simulink model "gnc_SpeedGovernor"  (R2026b)
settings: Solver=VariableStepAuto
values from neighbouring files (symbols this model uses):
  Ts = prm.Ts    [gnc_missionFSM.m]    (also in gnc_mpcPlantUpdate.m)
undefined symbols (not defined in the file or in its folder): P
libraries: sl_discontinuities x1, simulink x1
settings Model: Creator=aomar  LastModifiedBy=aomar

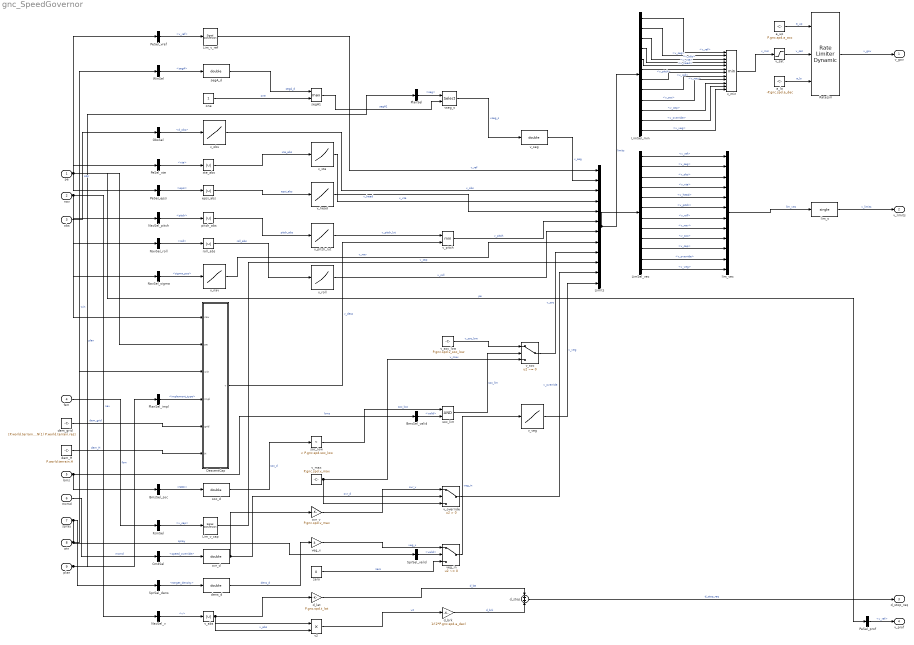
== system gnc_SpeedGovernor ==
  pe : Inport  OutDataTypeStr=Bus: Bus_PathError  SampleTime=Ts.gnc
  nav : Inport  Port=2  OutDataTypeStr=Bus: Bus_NavCond  SampleTime=Ts.gnc
  obs : Inport  Port=3  OutDataTypeStr=Bus: Bus_ObsFlags  SampleTime=Ts.gnc
  fsm : Inport  Port=4  OutDataTypeStr=Bus: Bus_FsmOut  SampleTime=Ts.gnc
  bms : Inport  Port=5  OutDataTypeStr=Bus: Bus_BmsStatus  SampleTime=Ts.gnc
  mcmd : Inport  Port=6  OutDataTypeStr=Bus: Bus_MissionCmd  SampleTime=Ts.gnc
  spray : Inport  Port=7  OutDataTypeStr=Bus: Bus_SprayDemand  SampleTime=Ts.gnc
  win : Inport  Port=8  OutDataTypeStr=Bus: Bus_PathWindow  SampleTime=Ts.gnc
  plan : Inport  Port=9  OutDataTypeStr=Bus: Bus_MissionPlan
  BmsSel_soc : BusSelector  OutputSignals=SOC
  BmsSel_valid : BusSelector  OutputSignals=valid
  CmdSel : BusSelector  OutputSignals=speed_override
  DescentCap : MATLAB Function  TreatAsAtomicUnit=on  mask{desc=P.gnc.desc}
  FsmSel : BusSelector  OutputSignals=v_cap
  LimSel_min : BusSelector  OutputSignals=v_ref,v_seg,v_obs,v_xte,v_head,v_pitch,v_roll,v_nav,v_soc,v_cap,v_override,v_veg
  LimSel_vec : BusSelector  OutputSignals=v_ref,v_seg,v_obs,v_xte,v_head,v_pitch,v_roll,v_nav,v_soc,v_cap,v_override,v_veg
  Lim_v_cap : SignalConversion  OverrideOpt=off
  Lim_v_ref : SignalConversion  OverrideOpt=off
  Limits : BusCreator  Inputs=12
  NavSel_pitch : BusSelector  OutputSignals=pitch
  NavSel_roll : BusSelector  OutputSignals=roll
  NavSel_sigma : BusSelector  OutputSignals=sigma_pos
  NavSel_v : BusSelector  OutputSignals=v
  ObsSel : BusSelector  OutputSignals=d_obs
  PeSel_epsi : BusSelector  OutputSignals=epsi
  PeSel_prof : BusSelector  OutputSignals=v_ref
  PeSel_vref : BusSelector  OutputSignals=v_ref
  PeSel_xte : BusSelector  OutputSignals=xte
  PlanSel : BusSelector  OutputSignals=seg
  PlanSel_impl : BusSelector  OutputSignals=implement_type
  RateLim : sl_discontinuities/Rate Limiter Dynamic
      settings: LibrarySourceBlock=|
      | simulink/Discontinuities/Rate Limiter
      | Dynamic
  SprSel_dens : BusSelector  OutputSignals=target_density
  SprSel_valid : BusSelector  OutputSignals=valid
  WinSel : BusSelector  OutputSignals=segA
  a_lo : Constant  Value=-P.gnc.spd.a_dec  OutDataTypeStr=double  SampleTime=Ts.gnc
  a_up : Constant  Value=P.gnc.spd.a_acc  OutDataTypeStr=double  SampleTime=Ts.gnc
  d_brk : Gain  Gain=1/(2*P.gnc.spd.a_dec)
  d_lat : Gain  Gain=P.gnc.spd.t_lat
  d_stop : Sum
  dem_H : Constant  Value=P.world.terrain.H  OutDataTypeStr=double
  dem_grid : Constant  Value=[P.world.terrain.xE(1) P.world.terrain.yN(1) P.world.terrain.res]  OutDataTypeStr=double
  dens_d : DataTypeConversion  OutDataTypeStr=double  RndMeth=Nearest
  epsi_abs : Abs  SaturateOnIntegerOverflow=off
  lim_s : DataTypeConversion  OutDataTypeStr=single  RndMeth=Nearest
  lim_vec : Mux  Inputs=12
  one : Constant  OutDataTypeStr=double  SampleTime=Ts.gnc
  ovr_d : DataTypeConversion  OutDataTypeStr=double  RndMeth=Nearest
  ovr_v : Gain  Gain=P.gnc.spd.v_max
  pitch_abs : Abs  SaturateOnIntegerOverflow=off
  roll_abs : Abs  SaturateOnIntegerOverflow=off
  segA1 : MinMax  Function=max  Inputs=2
  segA_d : DataTypeConversion  OutDataTypeStr=double  RndMeth=Nearest
  soc_d : DataTypeConversion  OutDataTypeStr=double  RndMeth=Nearest
  soc_lim : Logic  AllPortsSameDT=off  OutDataTypeStr=boolean
  soc_low : simulink/Logic and Bit Operations/Compare To Constant  relop=<  const=P.gnc.spd.soc_low  OutDataTypeStr=boolean
  v2 : Product  Inputs=**
  v_abs : Abs  SaturateOnIntegerOverflow=off
  v_head : Lookup_n-D  NumberOfTableDimensions=1  BreakpointsForDimension1=P.gnc.spd.head_x  Table=P.gnc.spd.head_v  ExtrapMethod=Clip  UseLastTableValue=on  InternalRulePriority=Speed  RndMeth=Simplest
  v_max : Constant  Value=P.gnc.spd.v_max  OutDataTypeStr=double  SampleTime=Ts.gnc
  v_min : MinMax  Inputs=12
  v_nav : Lookup_n-D  NumberOfTableDimensions=1  BreakpointsForDimension1=P.gnc.spd.nav_x  Table=P.gnc.spd.nav_v  ExtrapMethod=Clip  UseLastTableValue=on  InternalRulePriority=Speed  RndMeth=Simplest
  v_obs : Lookup_n-D  NumberOfTableDimensions=1  BreakpointsForDimension1=P.gnc.spd.obs_d  Table=P.gnc.spd.obs_v  ExtrapMethod=Clip  UseLastTableValue=on  InternalRulePriority=Speed  RndMeth=Simplest
  v_override : Switch  Criteria=u2 > Threshold  SaturateOnIntegerOverflow=off  InputSameDT=off
  v_pitch : MinMax  Inputs=2
  v_pitch_lut : Lookup_n-D  NumberOfTableDimensions=1  BreakpointsForDimension1=P.gnc.spd.pitch_x  Table=P.gnc.spd.pitch_v  ExtrapMethod=Clip  UseLastTableValue=on  InternalRulePriority=Speed  RndMeth=Simplest
  v_roll : Lookup_n-D  NumberOfTableDimensions=1  BreakpointsForDimension1=P.gnc.spd.roll_x  Table=P.gnc.spd.roll_v  ExtrapMethod=Clip  UseLastTableValue=on  InternalRulePriority=Speed  RndMeth=Simplest
  v_sat : Saturate  UpperLimit=P.gnc.spd.v_max  LowerLimit=0
  v_seg : DataTypeConversion  OutDataTypeStr=double  RndMeth=Nearest
  v_soc : Switch  Criteria=u2 ~= 0  SaturateOnIntegerOverflow=off  InputSameDT=off
  v_soc_low : Constant  Value=P.gnc.spd.v_soc_low  OutDataTypeStr=double  SampleTime=Ts.gnc
  v_veg : Lookup_n-D  NumberOfTableDimensions=1  BreakpointsForDimension1=P.gnc.spd.veg_x  Table=P.gnc.spd.veg_v  ExtrapMethod=Clip  UseLastTableValue=on  InternalRulePriority=Speed  RndMeth=Simplest
  v_xte : Lookup_n-D  NumberOfTableDimensions=1  BreakpointsForDimension1=P.gnc.spd.xte_x  Table=P.gnc.spd.xte_v  ExtrapMethod=Clip  UseLastTableValue=on  InternalRulePriority=Speed  RndMeth=Simplest
  veg_in : Switch  Criteria=u2 ~= 0  SaturateOnIntegerOverflow=off  InputSameDT=off
  veg_x : Gain  Gain=3
  vseg_s : Selector  NumberOfDimensions=2  InputPortWidth=3  IndexOptions=Index vector (port),Index vector (dialog)  Indices=1,4  OutputSizes=1
  xte_abs : Abs  SaturateOnIntegerOverflow=off
  zero : Constant  Value=0  OutDataTypeStr=double  SampleTime=Ts.gnc
  v_gov : Outport  OutDataTypeStr=double
  v_limits : Outport  Port=2  OutDataTypeStr=single
  d_stop_req : Outport  Port=3  OutDataTypeStr=double
  v_prof : Outport  Port=4  OutDataTypeStr=double
  wires:
  obs/1 -> ObsSel/1  "obs"
  fsm/1 -> FsmSel/1  "fsm"
  dem_grid/1 -> DescentCap/5(grid)  "dem_grid"
  dem_H/1 -> DescentCap/6(H)  "dem_H"
  bms/1 -> BmsSel_valid/1, BmsSel_soc/1  "bms"
  mcmd/1 -> CmdSel/1  "mcmd"
  spray/1 -> SprSel_dens/1, SprSel_valid/1  "spray"
  win/1 -> WinSel/1, DescentCap/3(win)  "win"
  plan/1 -> PlanSel/1, PlanSel_impl/1  "plan"
  PeSel_vref/1 -> Lim_v_ref/1  "<v_ref>"
  WinSel/1 -> segA_d/1  "<segA>"
  ObsSel/1 -> v_obs/1  "<d_obs>"
  PeSel_xte/1 -> xte_abs/1  "<xte>"
  PeSel_epsi/1 -> epsi_abs/1  "<epsi>"
  NavSel_pitch/1 -> pitch_abs/1  "<pitch>"
  NavSel_roll/1 -> roll_abs/1  "<roll>"
  NavSel_sigma/1 -> v_nav/1  "<sigma_pos>"
  PlanSel_impl/1 -> DescentCap/4(impl)  "<implement_type>"
  BmsSel_soc/1 -> soc_d/1  "<SOC>"
  FsmSel/1 -> Lim_v_cap/1  "<v_cap>"
  CmdSel/1 -> ovr_d/1  "<speed_override>"
  SprSel_dens/1 -> dens_d/1  "<target_density>"
  NavSel_v/1 -> v_abs/1  "<v>"
  one/1 -> segA1/2  "one"
  xte_abs/1 -> v_xte/1  "xte_abs"
  epsi_abs/1 -> v_head/1  "epsi_abs"
  pitch_abs/1 -> v_pitch_lut/1  "pitch_abs"
  roll_abs/1 -> v_roll/1  "roll_abs"
  v_abs/1 -> d_lat/1, v2/2, v2/1  "v_abs"
  Lim_v_ref/1 -> Limits/1  "v_ref"
  Lim_v_cap/1 -> Limits/10  "v_cap"
  v_obs/1 -> Limits/3  "v_obs"
  v_nav/1 -> Limits/8  "v_nav"
  DescentCap/1(v) -> v_pitch/2  "v_desc"
  segA_d/1 -> segA1/1  "segA_d"
  soc_d/1 -> soc_low/1  "soc_d"
  ovr_d/1 -> v_override/2, ovr_v/1  "ovr_d"
  dens_d/1 -> veg_x/1  "dens_d"
  segA1/1 -> vseg_s/2  "segA1"
  soc_low/1 -> soc_lim/1  "soc_low"
  v_max/1 -> v_soc/3, v_override/3  "v_max"
  ovr_v/1 -> v_override/1  "ovr_v"
  veg_x/1 -> veg_in/1  "veg_x"
  zero/1 -> veg_in/3  "zero"
  d_lat/1 -> d_stop/1  "d_lat"
  v2/1 -> d_brk/1  "v2"
  v_xte/1 -> Limits/4  "v_xte"
  v_head/1 -> Limits/5  "v_head"
  v_pitch_lut/1 -> v_pitch/1  "v_pitch_lut"
  v_roll/1 -> Limits/7  "v_roll"
  PlanSel/1 -> vseg_s/1  "<seg>"
  BmsSel_valid/1 -> soc_lim/2  "<valid>"
  SprSel_valid/1 -> veg_in/2  "<valid>"
  v_pitch/1 -> Limits/6  "v_pitch"
  v_soc_low/1 -> v_soc/1  "v_soc_low"
  soc_lim/1 -> v_soc/2  "soc_lim"
  d_brk/1 -> d_stop/2  "d_brk"
  vseg_s/1 -> v_seg/1  "vseg_s"
  v_override/1 -> Limits/11  "v_override"
  veg_in/1 -> v_veg/1  "veg_in"
  d_stop/1 -> d_stop_req/1  "d_stop_req"
  v_soc/1 -> Limits/9  "v_soc"
  v_veg/1 -> Limits/12  "v_veg"
  v_seg/1 -> Limits/2  "v_seg"
  Limits/1 -> LimSel_min/1, LimSel_vec/1  "limits"
  LimSel_min/1 -> v_min/1  "<v_ref>"
  LimSel_min/2 -> v_min/2  "<v_seg>"
  LimSel_min/3 -> v_min/3  "<v_obs>"
  LimSel_min/4 -> v_min/4  "<v_xte>"
  LimSel_min/5 -> v_min/5  "<v_head>"
  LimSel_min/6 -> v_min/6  "<v_pitch>"
  LimSel_min/7 -> v_min/7  "<v_roll>"
  LimSel_min/8 -> v_min/8  "<v_nav>"
  LimSel_min/9 -> v_min/9  "<v_soc>"
  LimSel_min/10 -> v_min/10  "<v_cap>"
  LimSel_min/11 -> v_min/11  "<v_override>"
  LimSel_min/12 -> v_min/12  "<v_veg>"
  LimSel_vec/1 -> lim_vec/1  "<v_ref>"
  LimSel_vec/2 -> lim_vec/2  "<v_seg>"
  LimSel_vec/3 -> lim_vec/3  "<v_obs>"
  LimSel_vec/4 -> lim_vec/4  "<v_xte>"
  LimSel_vec/5 -> lim_vec/5  "<v_head>"
  LimSel_vec/6 -> lim_vec/6  "<v_pitch>"
  LimSel_vec/7 -> lim_vec/7  "<v_roll>"
  LimSel_vec/8 -> lim_vec/8  "<v_nav>"
  LimSel_vec/9 -> lim_vec/9  "<v_soc>"
  LimSel_vec/10 -> lim_vec/10  "<v_cap>"
  LimSel_vec/11 -> lim_vec/11  "<v_override>"
  LimSel_vec/12 -> lim_vec/12  "<v_veg>"
  lim_vec/1 -> lim_s/1  "lim_vec"
  v_min/1 -> v_sat/1  "v_min"
  a_up/1 -> RateLim/1  "a_up"
  v_sat/1 -> RateLim/2  "v_sat"
  a_lo/1 -> RateLim/3  "a_lo"
  lim_s/1 -> v_limits/1  "v_limits"
  RateLim/1 -> v_gov/1  "v_gov"
  PeSel_prof/1 -> v_prof/1  "<v_ref>"
  pe/1 -> PeSel_prof/1, DescentCap/2(pe), PeSel_vref/1, PeSel_epsi/1, PeSel_xte/1  "pe"
  nav/1 -> NavSel_v/1, DescentCap/1(nav), NavSel_sigma/1, NavSel_roll/1, NavSel_pitch/1  "nav"

== matlab function gnc_SpeedGovernor/DescentCap ==
  settings: updateMethod=DISCRETE  sampleTime=Ts.gnc  description=Downhill speed limit: descent cap at the held nav pitch and along the path ahead (DEM look-ahead); body subsystems/gnc/gnc_descentLimit.m.
  data: nav input Bus: Bus_NavCond; v output double; pe input Bus: Bus_PathError; win input Bus: Bus_PathWindow; impl input; grid input; H input; desc parameter
function v = fcn(nav, pe, win, impl, grid, H, desc)
%#codegen
v = gnc_descentLimit(nav, pe, win, impl, grid, H, desc);
